simulink model "sm_car_"  (R2026b)
settings: Solver=ode23t  StopTime=100  MaxStep=0.4  AbsTol=1e-3  EnableMultiTasking=on
PreLoadFcn:
  | % Due to usability issue in Repeating Sequence block
  | warning('off','Simulink:Masking:Invalid');
  | 
  | % Eliminate unnecessary warnings in inactive variants
  | % Warnings generated only if you click through inactive variant
  | warning('off','MATLAB:nonExistentField');
  | warning('off','Simulink:Parameters:BlkParamUndefined');
PostLoadFcn:
  | set_param([bdroot '/Vehicle'],'popup_trailer','Off')
  | warning('off','sm:sli:setup:compile:LocalSolverNotSupported')
  | %sm_car_config_maneuver(bdroot,'WOT Braking');
  | sm_car_config_vehicle(bdroot,'false');
  | sm_car_config_logging(bdroot);
InitFcn:
  | sm_car_config_camera;
  | Vehicle = sm_car_vehcfg_checkConfig(Vehicle);
  | sm_car_check_tire_model(bdroot);
StartFcn:
  | tic;
StopFcn:
  | Elapsed_Sim_Time = toc;
  | % disp(['Elapsed Sim Time = ' num2str(Elapsed_Sim_Time)]);
undefined symbols (not defined in the file or in its folder): acc_theta, accel_ramp_rate, Axle1D, AxleIn, Camera, Control, Driver, Init, Maneuver, Pedal, Scene, ShaftL1, ShaftL2, ShaftR1, ShaftR2, Visual, X, xy_data_car_side, Y, Z
libraries: sm_lib x290, fl_lib x171, nesl_utility x144, simulink x60, simulink_extras x14, sdl_lib x14, SimscapeFluids_lib x7, Damper_Element x4, Tire_1x2x x4, ee_lib x3, Scene_Utilities x3, sharedTrackingLibrary x2
(part 11 of 22)

== system sm_car_/World/Scene/CRG Hockenheim F/STL Geometry Road ==
  Geometry : sm_lib/Body Elements/File Solid  ExtGeomFileName=CRG_Hockenheim_f.stl  UnitType=Custom  ExtGeomFileUnits=m  StepReaderType=HEX  ExportConvexHullGeometry=off  InertiaType=Custom  BasedOnType=DensityFromFile  Density=1000  DensityUnits=kg/m^3  Mass=1  MassUnits=kg  CenterOfMass=[0 0 0]  CenterOfMassUnits=m  MomentsOfInertia=[1 1 1]  MomentsOfInertiaUnits=kg*m^2  ProductsOfInertia=[0 0 0]  ProductsOfInertiaUnits=kg*m^2  GraphicType=FromGeometry  MarkerShape=Sphere  MarkerSize=10  GraphicVisPropType=SimpleVisualProperties  GraphicDiffuseColor=stl_clr  GraphicOpacity=stl_opc  GraphicSpecularColor=[0.5 0.5 0.5 1.0]  GraphicAmbientColor=[0.15 0.15 0.15 1.0]  GraphicEmissiveColor=[0.0 0.0 0.0 1.0]  GraphicShininess=75  DoExposeReferenceFrame=on  SerializedFrames=<Frames/>
  Transform Geometry : sm_lib/Frames and Transforms/Rigid Transform  RotationMethod=RotationSequence  FollAlignAxisA=+X  BaseAlignAxisA=+Y  FollAlignAxisB=+Y  BaseAlignAxisB=+Z  RotationStandardAxis=+Z  RotationAngle=0  RotationAngleUnits=rad  RotationArbitraryAxis=[0 0 1]  RotationSequenceAxes=FollowerAxes  RotationSequence=ZYX  RotationSequenceAngles=[stl_yaw stl_pitch stl_roll]  RotationSequenceAnglesUnits=rad  RotationMatrix=[1 0 0; 0 1 0; 0 0 1]  Quaternion=[1 0 0 0]  TranslationMethod=Cartesian  TranslationCartesianOffset=[stl_x stl_y stl_z]  TranslationCartesianOffsetUnits=m  TranslationStandardAxis=+Z  TranslationStandardOffset=0  TranslationStandardOffsetUnits=m  TranslationROffset=0  TranslationROffsetUnits=m  TranslationThetaOffset=0  TranslationThetaOffsetUnits=deg  TranslationZOffset=0  TranslationZOffsetUnits=m
  W : PMIOPort  Side=Right
  connections:
  Geometry/RConn1 -- Transform Geometry/RConn1
  Transform Geometry/LConn1 -- W/RConn1

== system sm_car_/World/Scene/Plane Grid/Grid ==
  Mesh Lines x : Subsystem  mask(Rectangular Mesh){mesh_lenx=grid_x, mesh_leny=grid_y, mesh_hx=hole_wy, mesh_hy=hole_ly, mesh_numhx=1, mesh_numhy=grid_num_sq_y, mesh_thickness=grid_z, mesh_rho=7000, mesh_color=grid_clr, mesh_opc=grid_opc}
      mask prompts: mesh_thickness "Thickness (m)"; mesh_rho "Density (kg/m^3)"; mesh_color "Color [RGB]"; mesh_opc "Opacity (0-1)"
      mask help: Rectangular mesh. Define outer dimensions, dimensions of holes, and thickness. R port is at the CG. Thickness defines the distance of the F frame from the B frame along the z-axis.
      mask init:
      | mesh_xsec = Extr_Data_Mesh(mesh_lenx, mesh_leny, mesh_numhx, mesh_numhy, mesh_hx, mesh_hy);
      mask DialogControl Control12 Prompt: Plot Profile
      mask DialogControl Control12 Callback:
      | v = get_param(gcb,'MaskWSVariables');
      | getMaskValue = containers.Map({v.Name}',{v.Value}');
      | evalin('base',...
      |     sprintf('Extr_Data_Mesh(%s,%s,%s,%s,%s,%s,''%s'');',...
      |     num2str(getMaskValue('mesh_lenx')),...
      |     num2str(getMaskValue('mesh_leny')),...
      |     num2str(getMaskValue('mesh_numhx')),...
      |     num2str(getMaskValue('mesh_numhy')),...
      |     num2str(getMaskValue('mesh_hx')),...
      |     num2str(getMaskValue('mesh_hy')),'plot'));
      mask DialogControl Control7 Prompt: X
      mask DialogControl Control8 Prompt: Y
      mask DialogControl Control9 Prompt: Mesh Length (m)
      mask DialogControl Control11 Prompt: Hole Length (m)
      mask DialogControl Control10 Prompt: Number of Holes
      mask Display: image('Mesh_IMAGE.png');
  "Mesh Lines y " : Subsystem  mask(Rectangular Mesh){mesh_lenx=grid_x, mesh_leny=grid_y, mesh_hx=hole_lx, mesh_hy=hole_wx, mesh_numhx=grid_num_sq_x, mesh_numhy=1, mesh_thickness=grid_z, mesh_rho=7000, mesh_color=grid_clr, mesh_opc=grid_opc}
      mask prompts: mesh_thickness "Thickness (m)"; mesh_rho "Density (kg/m^3)"; mesh_color "Color [RGB]"; mesh_opc "Opacity (0-1)"
      mask help: Rectangular mesh. Define outer dimensions, dimensions of holes, and thickness. R port is at the CG. Thickness defines the distance of the F frame from the B frame along the z-axis.
      mask init:
      | mesh_xsec = Extr_Data_Mesh(mesh_lenx, mesh_leny, mesh_numhx, mesh_numhy, mesh_hx, mesh_hy);
      mask DialogControl Control12 Prompt: Plot Profile
      mask DialogControl Control12 Callback:
      | v = get_param(gcb,'MaskWSVariables');
      | getMaskValue = containers.Map({v.Name}',{v.Value}');
      | evalin('base',...
      |     sprintf('Extr_Data_Mesh(%s,%s,%s,%s,%s,%s,''%s'');',...
      |     num2str(getMaskValue('mesh_lenx')),...
      |     num2str(getMaskValue('mesh_leny')),...
      |     num2str(getMaskValue('mesh_numhx')),...
      |     num2str(getMaskValue('mesh_numhy')),...
      |     num2str(getMaskValue('mesh_hx')),...
      |     num2str(getMaskValue('mesh_hy')),'plot'));
      mask DialogControl Control7 Prompt: X
      mask DialogControl Control8 Prompt: Y
      mask DialogControl Control9 Prompt: Mesh Length (m)
      mask DialogControl Control11 Prompt: Hole Length (m)
      mask DialogControl Control10 Prompt: Number of Holes
      mask Display: image('Mesh_IMAGE.png');
  Reference Frame{,1..3} (4 alike) : sm_lib/Frames and Transforms/Reference Frame
  R : PMIOPort  Side=Left
  connections:
  Reference Frame3/RConn1 -- Mesh Lines x/RConn2
  "Mesh Lines y "/LConn1 -- Mesh Lines x/LConn1 -- R/RConn1
  "Mesh Lines y "/RConn1 -- Reference Frame/RConn1
  Reference Frame1/RConn1 -- "Mesh Lines y "/RConn2
  Reference Frame2/RConn1 -- Mesh Lines x/RConn1

== system sm_car_/World/Scene/Plane Grid/Ground Plane ==
  Floor : sm_lib/Body Elements/Brick Solid  BrickDimensions=[gp_l, gp_w, gp_h]  BrickDimensionsUnits=m  ExportEntireGeometry=off  InertiaType=CalculateFromGeometry  BasedOnType=Density  Density=1000  DensityUnits=kg/m^3  Mass=1  MassUnits=kg  CenterOfMass=[0 0 0]  CenterOfMassUnits=m  MomentsOfInertia=[1 1 1]  MomentsOfInertiaUnits=kg*m^2  ProductsOfInertia=[0 0 0]  ProductsOfInertiaUnits=kg*m^2  GraphicType=FromGeometry  MarkerShape=Sphere  MarkerSize=10  GraphicVisPropType=SimpleVisualProperties  GraphicDiffuseColor=gp_clr  GraphicOpacity=gp_opc  GraphicSpecularColor=[0.5 0.5 0.5 1.0]  GraphicAmbientColor=[0.15 0.15 0.15 1.0]  GraphicEmissiveColor=[0.0 0.0 0.0 1.0]  GraphicShininess=75  DoExposeReferenceFrame=off  SerializedFrames=<Frames><Frame><Id>Frame1</Id><Value><Name>F</Name><Origin><Source>GeometricFeature</Source><FeatureName>+z surface</FeatureName></Origin><PrimaryAxis><DefinedDirection>+Z</DefinedDirection><Source>ReferenceFrame</Source><SourceDirection>+Z</SourceDirection><FeatureName></FeatureName></PrimaryAxis><SecondaryAxis><DefinedDirection>+X</DefinedDirection><Source>ReferenceFrame</Source><SourceDirection>+X</SourceDirection><FeatureName></FeatureName></SecondaryAxis></Value></Frame></Frames>
  W : PMIOPort  Side=Right
  connections:
  Floor/LConn1 -- W/RConn1

== system sm_car_/World/Scene/Skidpad/Circle Inner L ==
  Solid : sm_lib/Body Elements/Extruded Solid  ExtrusionType=General  PolygonNumSides=3  PolygonOuterRadius=1  PolygonOuterRadiusUnits=m  ExportEntireGeometry=off  ExtrusionCrossSection=xy_data_circ  ExtrusionCrossSectionUnits=m  ExportConvexHullGeometry=off  ExtrusionLength=circ_h  ExtrusionLengthUnits=m  InertiaType=CalculateFromGeometry  BasedOnType=Density  Density=1000  DensityUnits=kg/m^3  Mass=1  MassUnits=kg  CenterOfMass=[0 0 0]  CenterOfMassUnits=m  MomentsOfInertia=[1 1 1]  MomentsOfInertiaUnits=kg*m^2  ProductsOfInertia=[1 1 1]  ProductsOfInertiaUnits=kg*m^2  GraphicType=FromGeometry  MarkerShape=Sphere  MarkerSize=10  GraphicVisPropType=SimpleVisualProperties  GraphicDiffuseColor=[1.0 1.0 0.8]  GraphicOpacity=1.0  GraphicSpecularColor=[0.5 0.5 0.5 1.0]  GraphicAmbientColor=[0.15 0.15 0.15 1.0]  GraphicEmissiveColor=[0.0 0.0 0.0 1.0]  GraphicShininess=75  DoExposeReferenceFrame=on  SerializedFrames=<Frames/>
  W : PMIOPort  Side=Right
  connections:
  Solid/RConn1 -- W/RConn1

== system sm_car_/World/Scene/Skidpad/Circle Inner R ==
  Solid : sm_lib/Body Elements/Extruded Solid  ExtrusionType=General  PolygonNumSides=3  PolygonOuterRadius=1  PolygonOuterRadiusUnits=m  ExportEntireGeometry=off  ExtrusionCrossSection=xy_data_circ  ExtrusionCrossSectionUnits=m  ExportConvexHullGeometry=off  ExtrusionLength=circ_h  ExtrusionLengthUnits=m  InertiaType=CalculateFromGeometry  BasedOnType=Density  Density=1000  DensityUnits=kg/m^3  Mass=1  MassUnits=kg  CenterOfMass=[0 0 0]  CenterOfMassUnits=m  MomentsOfInertia=[1 1 1]  MomentsOfInertiaUnits=kg*m^2  ProductsOfInertia=[1 1 1]  ProductsOfInertiaUnits=kg*m^2  GraphicType=FromGeometry  MarkerShape=Sphere  MarkerSize=10  GraphicVisPropType=SimpleVisualProperties  GraphicDiffuseColor=[1.0 1.0 0.8]  GraphicOpacity=1.0  GraphicSpecularColor=[0.5 0.5 0.5 1.0]  GraphicAmbientColor=[0.15 0.15 0.15 1.0]  GraphicEmissiveColor=[0.0 0.0 0.0 1.0]  GraphicShininess=75  DoExposeReferenceFrame=on  SerializedFrames=<Frames/>
  W : PMIOPort  Side=Right
  connections:
  Solid/RConn1 -- W/RConn1

== system sm_car_/World/Scene/Skidpad/Circle Outer L ==
  Solid : sm_lib/Body Elements/Extruded Solid  ExtrusionType=General  PolygonNumSides=3  PolygonOuterRadius=1  PolygonOuterRadiusUnits=m  ExportEntireGeometry=off  ExtrusionCrossSection=xy_data_circ  ExtrusionCrossSectionUnits=m  ExportConvexHullGeometry=off  ExtrusionLength=circ_h  ExtrusionLengthUnits=m  InertiaType=CalculateFromGeometry  BasedOnType=Density  Density=1000  DensityUnits=kg/m^3  Mass=1  MassUnits=kg  CenterOfMass=[0 0 0]  CenterOfMassUnits=m  MomentsOfInertia=[1 1 1]  MomentsOfInertiaUnits=kg*m^2  ProductsOfInertia=[1 1 1]  ProductsOfInertiaUnits=kg*m^2  GraphicType=FromGeometry  MarkerShape=Sphere  MarkerSize=10  GraphicVisPropType=SimpleVisualProperties  GraphicDiffuseColor=[1.0 1.0 0.8]  GraphicOpacity=1.0  GraphicSpecularColor=[0.5 0.5 0.5 1.0]  GraphicAmbientColor=[0.15 0.15 0.15 1.0]  GraphicEmissiveColor=[0.0 0.0 0.0 1.0]  GraphicShininess=75  DoExposeReferenceFrame=on  SerializedFrames=<Frames/>
  W : PMIOPort  Side=Right
  connections:
  Solid/RConn1 -- W/RConn1

== system sm_car_/World/Scene/Skidpad/Circle Outer R ==
  Solid : sm_lib/Body Elements/Extruded Solid  ExtrusionType=General  PolygonNumSides=3  PolygonOuterRadius=1  PolygonOuterRadiusUnits=m  ExportEntireGeometry=off  ExtrusionCrossSection=xy_data_circ  ExtrusionCrossSectionUnits=m  ExportConvexHullGeometry=off  ExtrusionLength=circ_h  ExtrusionLengthUnits=m  InertiaType=CalculateFromGeometry  BasedOnType=Density  Density=1000  DensityUnits=kg/m^3  Mass=1  MassUnits=kg  CenterOfMass=[0 0 0]  CenterOfMassUnits=m  MomentsOfInertia=[1 1 1]  MomentsOfInertiaUnits=kg*m^2  ProductsOfInertia=[1 1 1]  ProductsOfInertiaUnits=kg*m^2  GraphicType=FromGeometry  MarkerShape=Sphere  MarkerSize=10  GraphicVisPropType=SimpleVisualProperties  GraphicDiffuseColor=[1.0 1.0 0.8]  GraphicOpacity=1.0  GraphicSpecularColor=[0.5 0.5 0.5 1.0]  GraphicAmbientColor=[0.15 0.15 0.15 1.0]  GraphicEmissiveColor=[0.0 0.0 0.0 1.0]  GraphicShininess=75  DoExposeReferenceFrame=on  SerializedFrames=<Frames/>
  W : PMIOPort  Side=Right
  connections:
  Solid/RConn1 -- W/RConn1

== system sm_car_/World/Scene/Skidpad/Ground Plane ==
  Floor : sm_lib/Body Elements/Brick Solid  BrickDimensions=[gp_l, gp_w, gp_h]  BrickDimensionsUnits=m  ExportEntireGeometry=off  InertiaType=CalculateFromGeometry  BasedOnType=Density  Density=1000  DensityUnits=kg/m^3  Mass=1  MassUnits=kg  CenterOfMass=[0 0 0]  CenterOfMassUnits=m  MomentsOfInertia=[1 1 1]  MomentsOfInertiaUnits=kg*m^2  ProductsOfInertia=[0 0 0]  ProductsOfInertiaUnits=kg*m^2  GraphicType=FromGeometry  MarkerShape=Sphere  MarkerSize=10  GraphicVisPropType=SimpleVisualProperties  GraphicDiffuseColor=gp_clr  GraphicOpacity=gp_opc  GraphicSpecularColor=[0.5 0.5 0.5 1.0]  GraphicAmbientColor=[0.15 0.15 0.15 1.0]  GraphicEmissiveColor=[0.0 0.0 0.0 1.0]  GraphicShininess=75  DoExposeReferenceFrame=off  SerializedFrames=<Frames><Frame><Id>Frame1</Id><Value><Name>F</Name><Origin><Source>GeometricFeature</Source><FeatureName>+z surface</FeatureName></Origin><PrimaryAxis><DefinedDirection>+Z</DefinedDirection><Source>ReferenceFrame</Source><SourceDirection>+Z</SourceDirection><FeatureName></FeatureName></PrimaryAxis><SecondaryAxis><DefinedDirection>+X</DefinedDirection><Source>ReferenceFrame</Source><SourceDirection>+X</SourceDirection><FeatureName></FeatureName></SecondaryAxis></Value></Frame></Frames>
  W : PMIOPort  Side=Right
  connections:
  Floor/LConn1 -- W/RConn1

== system sm_car_/Controller/Default/State Estimation/Sensor Noise Simulation/noise a_x ==
  <w> : Inport
  Add2 : Sum
  Band-Limited White Noise2 : simulink/Sources/Band-Limited White Noise  Cov=[1.22e-4]  Ts=0.01  seed=[512361]
  Quantizer2 : Quantizer  QuantizationInterval=0.0047
  Zero-Order Hold2 : ZeroOrderHold  SampleTime=0.01
  a_x_n : Outport
  wires:
  Add2/1 -> a_x_n/1  "a_x_n"
  <w>/1 -> Quantizer2/1
  Zero-Order Hold2/1 -> Add2/1
  Band-Limited White Noise2/1 -> Add2/2
  Quantizer2/1 -> Zero-Order Hold2/1

== system sm_car_/Controller/Default/State Estimation/Sensor Noise Simulation/noise a_y ==
  <w> : Inport
  Add2 : Sum
  Band-Limited White Noise2 : simulink/Sources/Band-Limited White Noise  Cov=[1.22e-4]  Ts=0.01  seed=[092756]
  Quantizer2 : Quantizer  QuantizationInterval=0.0047
  Zero-Order Hold2 : ZeroOrderHold  SampleTime=0.01
  a_y_n : Outport
  wires:
  Add2/1 -> a_y_n/1  "a_y_n"
  <w>/1 -> Quantizer2/1
  Zero-Order Hold2/1 -> Add2/1
  Band-Limited White Noise2/1 -> Add2/2
  Quantizer2/1 -> Zero-Order Hold2/1

== system sm_car_/Controller/Default/State Estimation/Sensor Noise Simulation/noise omega_fl ==
  <w> : Inport
  Add2 : Sum
  Band-Limited White Noise2 : simulink/Sources/Band-Limited White Noise  Cov=[1e-4]  Ts=0.01  seed=[12451]
  Quantizer2 : Quantizer  QuantizationInterval=2 * pi / 25
  Zero-Order Hold2 : ZeroOrderHold  SampleTime=0.01
  omega_rl : Outport
  wires:
  Add2/1 -> omega_rl/1  "omega_rl"
  <w>/1 -> Quantizer2/1
  Zero-Order Hold2/1 -> Add2/1
  Band-Limited White Noise2/1 -> Add2/2
  Quantizer2/1 -> Zero-Order Hold2/1

== system sm_car_/Controller/Default/State Estimation/Sensor Noise Simulation/noise omega_fr ==
  <w> : Inport
  Add3 : Sum
  Band-Limited White Noise3 : simulink/Sources/Band-Limited White Noise  Cov=[1e-4]  Ts=0.01  seed=[68595]
  Quantizer3 : Quantizer  QuantizationInterval=2 * pi / 25
  Zero-Order Hold3 : ZeroOrderHold  SampleTime=0.01
  omega_rr : Outport
  wires:
  Add3/1 -> omega_rr/1  "omega_rr"
  Band-Limited White Noise3/1 -> Add3/2
  Zero-Order Hold3/1 -> Add3/1
  <w>/1 -> Quantizer3/1
  Quantizer3/1 -> Zero-Order Hold3/1

== system sm_car_/Controller/Default/State Estimation/Sensor Noise Simulation/noise omega_rl ==
  <w> : Inport
  Add : Sum
  Band-Limited White Noise : simulink/Sources/Band-Limited White Noise  Cov=[1e-4]  Ts=0.01  seed=[23341]
  Quantizer : Quantizer  QuantizationInterval=2 * pi / 94
  Zero-Order Hold : ZeroOrderHold  SampleTime=0.01
  omega_rl : Outport
  wires:
  Quantizer/1 -> Zero-Order Hold/1
  <w>/1 -> Quantizer/1
  Band-Limited White Noise/1 -> Add/2
  Add/1 -> omega_rl/1  "omega_rl"
  Zero-Order Hold/1 -> Add/1

== system sm_car_/Controller/Default/State Estimation/Sensor Noise Simulation/noise omega_rr ==
  <w> : Inport
  Add1 : Sum
  Band-Limited White Noise1 : simulink/Sources/Band-Limited White Noise  Cov=[1e-4]  Ts=0.01  seed=[41245]
  Quantizer1 : Quantizer  QuantizationInterval=2 * pi / 94
  Zero-Order Hold1 : ZeroOrderHold  SampleTime=0.01
  omega_rr : Outport
  wires:
  Add1/1 -> omega_rr/1  "omega_rr"
  Quantizer1/1 -> Zero-Order Hold1/1
  <w>/1 -> Quantizer1/1
  Band-Limited White Noise1/1 -> Add1/2
  Zero-Order Hold1/1 -> Add1/1

== system sm_car_/Controller/Default/State Estimation/Sensor Noise Simulation/noise v_gps ==
  <vx> : Inport
  <vy> : Inport  Port=2
  <vz> : Inport  Port=3
  Add : Sum  Inputs=+++
  Add2 : Sum
  Band-Limited White Noise2 : simulink/Sources/Band-Limited White Noise  Cov=[9e-4]  Ts=0.1  seed=[645743]
  Quantizer2 : Quantizer  QuantizationInterval=0.01
  Sqrt : Sqrt
  Square : Math  Operator=square
  Square1 : Math  Operator=square
  Square2 : Math  Operator=square
  Zero-Order Hold2 : ZeroOrderHold  SampleTime=0.1
  V_n : Outport
  wires:
  Quantizer2/1 -> Zero-Order Hold2/1
  Band-Limited White Noise2/1 -> Add2/2
  Zero-Order Hold2/1 -> Add2/1
  <vx>/1 -> Square/1
  Add2/1 -> V_n/1  "V_n"
  Square/1 -> Add/1
  <vy>/1 -> Square1/1
  <vz>/1 -> Square2/1
  Square1/1 -> Add/2
  Square2/1 -> Add/3
  Add/1 -> Sqrt/1
  Sqrt/1 -> Quantizer2/1

== system sm_car_/Controller/Default/State Estimation/Sensor Noise Simulation/noise yaw rate ==
  <w> : Inport
  Add2 : Sum
  Band-Limited White Noise2 : simulink/Sources/Band-Limited White Noise  Cov=[7.29e-7]  Ts=0.01  seed=[809953]
  Quantizer2 : Quantizer  QuantizationInterval=0.001
  Zero-Order Hold2 : ZeroOrderHold  SampleTime=0.01
  nYaw_n : Outport
  wires:
  Quantizer2/1 -> Zero-Order Hold2/1
  Band-Limited White Noise2/1 -> Add2/2
  Zero-Order Hold2/1 -> Add2/1
  <w>/1 -> Quantizer2/1
  Add2/1 -> nYaw_n/1  "nYaw_n"

== system sm_car_/Controller/TrqVec 4Motor/Brake Control/ABS/Calculate Slip ==
  WhlSpd : Inport
  VehSpdEst : Inport  Port=2
  Abs : Abs  ZeroCross=off  SaturateOnIntegerOverflow=off
  Bus Creator : BusCreator  Inputs=4
  Bus Selector1 : BusSelector  OutputSignals=L1.v,R1.v,L2.v,R2.v
  Constant : Constant
  Demux : Demux
  Fcn{,1..3} (4 alike) : Fcn  Expr=abs(u(1)*u(2)-u(3))/u(3)
  Mux{,1..3} (4 alike) : Mux  Inputs=3
  Mux4 : Mux
  Mux5 : Mux
  Product : Product
  Saturation : Saturate  UpperLimit=inf  LowerLimit=eps  ZeroCross=off
  Saturation1 : Saturate  UpperLimit=1  LowerLimit=0
  Sign : Signum  ZeroCross=off
  Wheel Speeds and Slip : Scope  NumInputPorts=2
      settings: ActiveDisplayYMinimum=-11.64241  ActiveDisplayYMaximum=114.01232  DataLoggingVariableName=ScopeData2
  Slip : Outport  VectorParamsAs1DForOutWhenUnconnected=off
  wires:
  WhlSpd/1 -> Bus Selector1/1
  Bus Selector1/2 -> Mux4/2, Mux1/2  "<v>"
  Bus Selector1/4 -> Mux4/4, Mux3/2  "<v>"
  Bus Selector1/1 -> Mux4/1, Mux/2  "<v>"
  Bus Selector1/3 -> Mux4/3, Mux2/2  "<v>"
  Constant/1 -> Mux/1, Mux1/1, Mux3/1, Mux2/1
  VehSpdEst/1 -> Sign/1, Abs/1
  Demux/1 -> Bus Creator/1  "L1"
  Demux/2 -> Bus Creator/2  "R1"
  Demux/3 -> Bus Creator/3  "L2"
  Demux/4 -> Bus Creator/4  "R2"
  Bus Creator/1 -> Wheel Speeds and Slip/2, Slip/1  "Slip"
  Product/1 -> Mux3/3, Mux2/3, Mux1/3, Mux/3
  Abs/1 -> Saturation/1
  Saturation/1 -> Product/1
  Sign/1 -> Product/2
  Mux/1 -> Fcn/1
  Mux1/1 -> Fcn1/1
  Mux2/1 -> Fcn2/1
  Mux3/1 -> Fcn3/1
  Mux4/1 -> Wheel Speeds and Slip/1  "Wheel Speeds"
  Mux5/1 -> Saturation1/1
  Saturation1/1 -> Demux/1
  Fcn/1 -> Mux5/1  "L1"
  Fcn1/1 -> Mux5/2  "R1"
  Fcn2/1 -> Mux5/3  "L2"
  Fcn3/1 -> Mux5/4  "R2"

== system sm_car_/Controller/TrqVec 4Motor/Brake Control/ABS/Sensor ==
  Body : Inport
  WhlSpd : Inport  Port=2
  Bus Creator{,3..5} (4 alike) : BusCreator  Inputs=1
  Bus Creator6 : BusCreator  Inputs=5
  Bus Selector : BusSelector  OutputSignals=vx,vy  OutputAsBus=on
  Bus Selector4 : BusSelector  OutputSignals=WhlL1.n,WhlR1.n,WhlL2.n,WhlR2.n,WhlL2.qxyz
  Gain : Gain  Gain=3.6*abs_tire_radiusF
  Gain1 : Gain  Gain=3.6*abs_tire_radiusF
  Gain2 : Gain  Gain=3.6*abs_tire_radiusR
  Gain3 : Gain  Gain=3.6*abs_tire_radiusR
  Gain4 : Gain  Gain=3.6
  Terminator1 : Terminator  Commented=on
  Vel in xy plane : Fcn  Expr=sqrt(u(1)^2+u(2)^2)
  missing tooth : Subsystem  Commented=on
  GroundSpd : Outport  VectorParamsAs1DForOutWhenUnconnected=off
  wires:
  Gain1/1 -> Bus Creator3/1  "v"
  missing tooth/1(Out1) -> Terminator1/1  "v"
  Gain2/1 -> Bus Creator4/1  "v"
  Bus Selector4/5 -> missing tooth/2(<qxyz>)  "<qxyz>"
  Bus Creator5/1 -> Bus Creator6/5  "R2"
  Gain3/1 -> Bus Creator5/1  "v"
  Bus Creator/1 -> Bus Creator6/2  "L1"
  Bus Selector4/2 -> Gain1/1  "<n>"
  Bus Creator4/1 -> Bus Creator6/4  "L2"
  Bus Selector4/3 -> Gain2/1, missing tooth/1(<omega>)  "<n>"
  Gain/1 -> Bus Creator/1  "v"
  Body/1 -> Bus Selector/1
  Bus Creator3/1 -> Bus Creator6/3  "R1"
  Gain4/1 -> Bus Creator6/1  "v"
  Bus Selector4/1 -> Gain/1  "<n>"
  Bus Selector4/4 -> Gain3/1  "<n>"
  WhlSpd/1 -> Bus Selector4/1
  Bus Creator6/1 -> GroundSpd/1
  Vel in xy plane/1 -> Gain4/1  "speed"
  Bus Selector/1 -> Vel in xy plane/1

== system sm_car_/Controller/TrqVec 4Motor/Brake Control/ABS/Valve Control L1 ==
  Slip : Inport
  vSpdEst : Inport  Port=2
  Categorize Surface : Subsystem
  Code to Valves : Subsystem
  Demux : Demux  Outputs=2
  Logic : Stateflow chart  TreatAsAtomicUnit=on
  Mux : Mux  Inputs=2
  Product : Product
  Subsystem : Subsystem
  Subsystem1 : Subsystem
  Valve : Outport  VectorParamsAs1DForOutWhenUnconnected=off
  wires:
  Logic/1(Mod_State) -> Categorize Surface/1(Mod State), Code to Valves/1(C)
  Logic/2(Mod_Dur) -> Product/2
  Slip/1 -> Logic/1(Slip)
  Code to Valves/1(V) -> Product/1
  vSpdEst/1 -> Logic/2(vSpdEst)
  Product/1 -> Demux/1
  Demux/1 -> Subsystem/1(OnT)
  Demux/2 -> Subsystem1/1(OnT)
  Mux/1 -> Valve/1
  Subsystem/1(vSig) -> Mux/1, Categorize Surface/2(Apply Valve)
  Subsystem1/1(vSig) -> Mux/2

== system sm_car_/Controller/TrqVec 4Motor/Brake Control/ABS/Valve Control L2 ==
  Slip : Inport
  vSpdEst : Inport  Port=2
  Categorize Surface : Subsystem
  Code to Valves : Subsystem
  Demux : Demux  Outputs=2
  Logic : Stateflow chart  TreatAsAtomicUnit=on
  Mux : Mux  Inputs=2
  Product : Product
  Subsystem : Subsystem
  Subsystem1 : Subsystem
  Valve : Outport  VectorParamsAs1DForOutWhenUnconnected=off
  wires:
  Logic/1(Mod_State) -> Categorize Surface/1(Mod State), Code to Valves/1(C)
  Logic/2(Mod_Dur) -> Product/2
  Slip/1 -> Logic/1(Slip)
  Code to Valves/1(V) -> Product/1
  vSpdEst/1 -> Logic/2(vSpdEst)
  Product/1 -> Demux/1
  Demux/1 -> Subsystem/1(OnT)
  Demux/2 -> Subsystem1/1(OnT)
  Mux/1 -> Valve/1
  Subsystem/1(vSig) -> Mux/1, Categorize Surface/2(Apply Valve)
  Subsystem1/1(vSig) -> Mux/2

== system sm_car_/Controller/TrqVec 4Motor/Brake Control/ABS/Valve Control R1 ==
  Slip : Inport
  vSpdEst : Inport  Port=2
  Categorize Surface : Subsystem
  Code to Valves : Subsystem
  Demux : Demux  Outputs=2
  Logic : Stateflow chart  TreatAsAtomicUnit=on
  Mux : Mux  Inputs=2
  Product : Product
  Subsystem : Subsystem
  Subsystem1 : Subsystem
  Valve : Outport  VectorParamsAs1DForOutWhenUnconnected=off
  wires:
  Logic/1(Mod_State) -> Categorize Surface/1(Mod State), Code to Valves/1(C)
  Logic/2(Mod_Dur) -> Product/2
  Slip/1 -> Logic/1(Slip)
  Code to Valves/1(V) -> Product/1
  vSpdEst/1 -> Logic/2(vSpdEst)
  Product/1 -> Demux/1
  Demux/1 -> Subsystem/1(OnT)
  Demux/2 -> Subsystem1/1(OnT)
  Mux/1 -> Valve/1
  Subsystem/1(vSig) -> Mux/1, Categorize Surface/2(Apply Valve)
  Subsystem1/1(vSig) -> Mux/2

== system sm_car_/Controller/TrqVec 4Motor/Brake Control/ABS/Valve Control R2 ==
  Slip : Inport
  vSpdEst : Inport  Port=2
  Categorize Surface : Subsystem
  Code to Valves : Subsystem
  Demux : Demux  Outputs=2
  Logic : Stateflow chart  TreatAsAtomicUnit=on
  Mux : Mux  Inputs=2
  Product : Product
  Subsystem : Subsystem
  Subsystem1 : Subsystem
  Valve : Outport  VectorParamsAs1DForOutWhenUnconnected=off
  wires:
  Logic/1(Mod_State) -> Categorize Surface/1(Mod State), Code to Valves/1(C)
  Logic/2(Mod_Dur) -> Product/2
  Slip/1 -> Logic/1(Slip)
  Code to Valves/1(V) -> Product/1
  vSpdEst/1 -> Logic/2(vSpdEst)
  Product/1 -> Demux/1
  Demux/1 -> Subsystem/1(OnT)
  Demux/2 -> Subsystem1/1(OnT)
  Mux/1 -> Valve/1
  Subsystem/1(vSig) -> Mux/1, Categorize Surface/2(Apply Valve)
  Subsystem1/1(vSig) -> Mux/2

== system sm_car_/Controller/TrqVec 4Motor/Brake Control/ABS/Vehicle Speed ==
  Sensors : Inport
  Bus Selector : BusSelector  OutputSignals=v
  vSpdEst : Outport  VectorParamsAs1DForOutWhenUnconnected=off
  wires:
  Sensors/1 -> Bus Selector/1
  Bus Selector/1 -> vSpdEst/1  "<v>"

== system sm_car_/Controller/TrqVec 4Motor/Power_TqVec/Torque Vectoring/Accel Torque Request ==
  note: Assumes both rear motors have same torque speed curve
  MotSpdL2 : Inport
  MotSpdR2 : Inport  Port=2
  MaxMotTrqVsSpdA1 : Lookup_n-D  NumberOfTableDimensions=1  BreakpointsForDimension1=Control.MotorL2.TorqueSpd.w.Value  Table=Control.MotorL2.TorqueSpd.trq.Value  ExtrapMethod=Clip  UseLastTableValue=on  InternalRulePriority=Speed  OutDataTypeStr=Inherit: Inherit from 'Table data'  RndMeth=Simplest
  Terminator : Terminator
  rads_to_rpm : Gain  Gain=30/pi
  rads_to_rpm1 : Gain  Gain=30/pi
  TrqMax : Outport  VectorParamsAs1DForOutWhenUnconnected=off
  wires:
  rads_to_rpm1/1 -> Terminator/1
  MotSpdR2/1 -> rads_to_rpm1/1
  MaxMotTrqVsSpdA1/1 -> TrqMax/1
  MotSpdL2/1 -> rads_to_rpm/1
  rads_to_rpm/1 -> MaxMotTrqVsSpdA1/1

== system sm_car_/Controller/TrqVec 4Motor/Power_TqVec/Torque Vectoring/Enable ==
  note: Ramp up amount of torque vectoring over a range.
  note: Steer angle threshold to enable torque vectoring
  vx : Inport
  aSteerWheel : Inport  Port=2
  Abs : Abs  ZeroCross=off  SaturateOnIntegerOverflow=off
  Data Type Conversion : DataTypeConversion  OutDataTypeStr=double  SaturateOnIntegerOverflow=off  RndMeth=Floor
  Divide : Product  Inputs=*/
  Enable vx : simulink/Logic and Bit Operations/Compare To Constant  relop=>  const=vx_enable  OutDataTypeStr=boolean  ZeroCross=off
  Gain : Gain  Gain=0.25
  Product : Product
  Saturation : Saturate  UpperLimit=1  LowerLimit=0  ZeroCross=off
  Subtract : Sum  Inputs=+-
  const : Constant  Value=aSteerWheel_enable
  Enable : Outport  VectorParamsAs1DForOutWhenUnconnected=off
  wires:
  Gain/1 -> Divide/1
  Product/1 -> Enable/1
  Divide/1 -> Saturation/1
  Subtract/1 -> Gain/1
  Abs/1 -> Subtract/1
  Saturation/1 -> Product/2
  Data Type Conversion/1 -> Product/1
  Enable vx/1 -> Data Type Conversion/1
  const/1 -> Subtract/2, Divide/2
  aSteerWheel/1 -> Abs/1
  vx/1 -> Enable vx/1

== system sm_car_/Controller/TrqVec 4Motor/Power_TqVec/Torque Vectoring/Vehicle Slip Angle Error ==
  vx : Inport
  aSteerWheel : Inport  Port=2
  nYaw : Inport  Port=3
  Add1 : Sum  Inputs=-+
  Distance Yaw Ctr Front Axle : Constant  Value=Vehicle.Chassis.Body.sAxle2.Value(1)/(-2)
  Divide3 : Product  Inputs=*/
  Multiply2 : Product
  Mux : Mux  Inputs=2
  Scope : Scope  NumInputPorts=2
      settings: ActiveDisplayYMinimum=-0.04829  ActiveDisplayYMaximum=0.00545
  Steering Wheel to Driving Wheel : Gain  Gain=aStr_to_aWhl
  Error : Outport  VectorParamsAs1DForOutWhenUnconnected=off
  wires:
  Mux/1 -> Scope/1
  Multiply2/1 -> Divide3/1
  Steering Wheel to Driving Wheel/1 -> Mux/2, Add1/2  "Wheel Angle"
  Distance Yaw Ctr Front Axle/1 -> Multiply2/1
  aSteerWheel/1 -> Steering Wheel to Driving Wheel/1
  nYaw/1 -> Multiply2/2
  Add1/1 -> Scope/2, Error/1  "Error"
  vx/1 -> Divide3/2
  Divide3/1 -> Add1/1, Mux/1  "Vehicle Slip Angle"

== system sm_car_/Controller/TrqVec_FLC_V3/Power Control/State Estimation/Sensor Noise Simulation ==
  <vx> : Inport
  <vy> : Inport  Port=2
  <vz> : Inport  Port=3
  <nYaw> : Inport  Port=4
  <gx> : Inport  Port=5
  <gy> : Inport  Port=6
  <w_fl> : Inport  Port=7
  <w_fr> : Inport  Port=8
  <w_rl> : Inport  Port=9
  <w_rr> : Inport  Port=10
  delta : Inport  Port=11
  Bus Creator : BusCreator  Inputs=5
  Bus Creator1 : BusCreator  Inputs=4
  Data Type Conversion{,3..10} (9 alike) : DataTypeConversion  OutDataTypeStr=single  SaturateOnIntegerOverflow=off  RndMeth=Floor
  noise a_x : Subsystem
  noise a_y : Subsystem
  noise omega_fl : Subsystem
  noise omega_fr : Subsystem
  noise omega_rl : Subsystem
  noise omega_rr : Subsystem
  noise v_gps : Subsystem
  noise yaw rate : Subsystem
  Inputs : Outport
  Meas : Outport  Port=2
  wires:
  <vz>/1 -> noise v_gps/3(<vz>)
  <vy>/1 -> noise v_gps/2(<vy>)
  noise v_gps/1(V_n) -> Data Type Conversion/1
  Data Type Conversion10/1 -> Bus Creator/5  "omega_rr_n"
  Data Type Conversion9/1 -> Bus Creator/4  "omega_rl_n"
  Data Type Conversion8/1 -> Bus Creator/1  "delta"
  Data Type Conversion7/1 -> Bus Creator/3  "omega_fr_n"
  Data Type Conversion6/1 -> Bus Creator/2  "omega_fl_n"
  Data Type Conversion5/1 -> Bus Creator1/4  "a_y_n"
  Data Type Conversion4/1 -> Bus Creator1/3  "a_x_n"
  Data Type Conversion3/1 -> Bus Creator1/2  "nYaw_n"
  Data Type Conversion/1 -> Bus Creator1/1  "V_GPS_n"
  Bus Creator1/1 -> Meas/1
  noise omega_fr/1(omega_rr) -> Data Type Conversion7/1
  <w_rr>/1 -> noise omega_rr/1(<w>)
  noise omega_rr/1(omega_rr) -> Data Type Conversion10/1
  <gy>/1 -> noise a_y/1(<w>)
  <w_rl>/1 -> noise omega_rl/1(<w>)
  noise yaw rate/1(nYaw_n) -> Data Type Conversion3/1
  noise omega_rl/1(omega_rl) -> Data Type Conversion9/1
  Bus Creator/1 -> Inputs/1
  noise a_y/1(a_y_n) -> Data Type Conversion5/1
  noise omega_fl/1(omega_rl) -> Data Type Conversion6/1
  <vx>/1 -> noise v_gps/1(<vx>)
  noise a_x/1(a_x_n) -> Data Type Conversion4/1
  <gx>/1 -> noise a_x/1(<w>)
  <w_fr>/1 -> noise omega_fr/1(<w>)
  <nYaw>/1 -> noise yaw rate/1(<w>)
  <w_fl>/1 -> noise omega_fl/1(<w>)
  delta/1 -> Data Type Conversion8/1

== system sm_car_/Controller/TrqVec_FLC_V3/Power Control/State Estimation/UKF ==
  StateTransitionFcnInputs : Inport  PortDimensions=5
  y1 : Inport  Port=2
  Compare To Constant : simulink/Logic and Bit Operations/Compare To Constant  relop=<=  const=0.5  OutDataTypeStr=boolean
  Constant : Constant  Value=0  OutDataTypeStr=single  SampleTime=0.003
  Constant1 : Constant  Value=0  OutDataTypeStr=single
  Delay : Delay  DelayLength=1  SampleTime=0.003
  Demux : Demux  Outputs=5
  MATLAB Function : MATLAB Function  TreatAsAtomicUnit=on
  Mux : Mux  Inputs=5
  Switch : Switch  Criteria=u2 ~= 0  SaturateOnIntegerOverflow=off  InputSameDT=off
  Unscented Kalman Filter : sharedTrackingLibrary/Unscented Kalman Filter  StateTransitionFcn=prediction_model  HasAdditiveProcessNoise=Additive  ProcessNoise=diag([1e-5, 8e-6, 1e-6, 5e-5, 1e-4])  HasTimeVaryingProcessNoise=on  HasStateTransitionFcnExtraArgument=1  InitialState=[0.4; 0; 0; 0; 0]  InitialStateCovariance=diag([0.04, 0.04, 1e-3, 0.1, 0.1])  Alpha=0.1  Beta=2  Kappa=0  MeasurementFcn1=measurement_model  HasMeasurementEnablePort1=off  HasAdditiveMeasurementNoise1=Additive  MeasurementNoise1=[9e-4, 7.29e-7, 1.22e-4, 1.22e-4]  HasTimeVaryingMeasurementNoise1=off  HasMeasurementFcnExtraArgument1=1  HasMeasurementWrapping1=on  MeasurementFcn2=myMeasurementFcn  HasMeasurementEnablePort2=off  HasAdditiveMeasurementNoise2=Additive  MeasurementNoise2=1  HasTimeVaryingMeasurementNoise2=off  HasMeasurementFcnExtraArgument2=0  HasMeasurementWrapping2=off  MeasurementFcn3=myMeasurementFcn  HasMeasurementEnablePort3=off  HasAdditiveMeasurementNoise3=Additive  MeasurementNoise3=1  HasTimeVaryingMeasurementNoise3=off  HasMeasurementFcnExtraArgument3=0  HasMeasurementWrapping3=off  MeasurementFcn4=myMeasurementFcn  HasMeasurementEnablePort4=off  HasAdditiveMeasurementNoise4=Additive  MeasurementNoise4=1  HasTimeVaryingMeasurementNoise4=off  HasMeasurementFcnExtraArgument4=0  HasMeasurementWrapping4=off  MeasurementFcn5=myMeasurementFcn  HasMeasurementEnablePort5=off  HasAdditiveMeasurementNoise5=Additive  MeasurementNoise5=1  HasTimeVaryingMeasurementNoise5=off  HasMeasurementFcnExtraArgument5=0  HasMeasurementWrapping5=off  EnableMultirate=off  StateTransitionFcnSampleTime=1  MeasurementFcn1SampleTime=1  MeasurementFcn2SampleTime=1  MeasurementFcn3SampleTime=1  MeasurementFcn4SampleTime=1  MeasurementFcn5SampleTime=1  UseCurrentEstimator=on  OutputStateCovariance=off  DataType=single  SampleTime=0.003  NumberOfMeasurements=1
      settings: LibrarySourceBlock=cstblocks/State Estimation/Unscented Kalman Filter
  xhat : Outport
  wires:
  Mux/1 -> xhat/1
  Demux/5 -> Mux/5
  Demux/4 -> Mux/4
  Demux/3 -> Mux/3
  Switch/1 -> Mux/2
  Demux/2 -> Switch/3
  Demux/1 -> Compare To Constant/1, Mux/1
  Constant1/1 -> Switch/1
  Compare To Constant/1 -> Switch/2
  Delay/1 -> MATLAB Function/1(xhat)
  MATLAB Function/1(Q) -> Unscented Kalman Filter/1
  Unscented Kalman Filter/1 -> Demux/1, Delay/1
  Constant/1 -> Unscented Kalman Filter/4
  StateTransitionFcnInputs/1 -> Unscented Kalman Filter/2
  y1/1 -> Unscented Kalman Filter/3

== system sm_car_/Driver/Closed Loop/Maneuver/Count Lap/Triggered Subsystem ==
  Up Down : Inport
  Trigger : TriggerPort  VariantControl=Variant  ZeroCross=off
  Memory : Memory  InheritSampleTime=on
  Sum : Sum  Inputs=|++
  Num Laps : Outport  VectorParamsAs1DForOutWhenUnconnected=off
  wires:
  Memory/1 -> Sum/1
  Sum/1 -> Memory/1, Num Laps/1
  Up Down/1 -> Sum/2

== system sm_car_/Driver/Closed Loop/Maneuver/PoseTargetVisual/Count Lap ==
  note: If on the previous step, the vehicle was in the last 5 percent of the trajectory and now it is on the first 5 percent of the trajectory, increment the number of laps.
  note: If on the previous step, the vehicle was in the first 5 percent of the trajectory and now it is on the last 5 percent of the trajectory, decrement the number of laps.
  ad : Inport
  AND Add Lap : Logic  IconShape=distinctive  AllPortsSameDT=off  OutDataTypeStr=boolean
  AND Subtract Lap : Logic  IconShape=distinctive  AllPortsSameDT=off  OutDataTypeStr=boolean
  Data Type Conversion : DataTypeConversion  SaturateOnIntegerOverflow=off  RndMeth=Floor
  Data Type Conversion1 : DataTypeConversion  SaturateOnIntegerOverflow=off  RndMeth=Floor
  First 5 Percent : simulink/Logic and Bit Operations/Compare To Constant  relop=<=  const=max(Maneuver.Trajectory.xTrajectory.Value)*0.05  OutDataTypeStr=boolean  ZeroCross=off
  Last 5 Percent : simulink/Logic and Bit Operations/Compare To Constant  relop=>=  const=max(Maneuver.Trajectory.xTrajectory.Value)*0.95  OutDataTypeStr=boolean  ZeroCross=off
  Memory : Memory  InitialCondition=false
  Memory2 : Memory  InitialCondition=false
  OR : Logic  Operator=OR  IconShape=distinctive  AllPortsSameDT=off  OutDataTypeStr=boolean
  Sum : Sum  Inputs=+-|
  Triggered Subsystem : Subsystem  TreatAsAtomicUnit=on
  Lap Count : Outport  VectorParamsAs1DForOutWhenUnconnected=off
  wires:
  Data Type Conversion1/1 -> Sum/2
  Data Type Conversion/1 -> Sum/1
  ad/1 -> First 5 Percent/1, Last 5 Percent/1
  Last 5 Percent/1 -> AND Subtract Lap/2, Memory/1  "Last 5"
  Triggered Subsystem/1(Num Laps) -> Lap Count/1
  First 5 Percent/1 -> Memory2/1, AND Add Lap/2  "First 5"
  Memory/1 -> AND Add Lap/1
  OR/1 -> Triggered Subsystem/Trigger  "Trigger"
  Memory2/1 -> AND Subtract Lap/1
  AND Add Lap/1 -> Data Type Conversion/1, OR/1  "Add Lap"
  AND Subtract Lap/1 -> OR/2, Data Type Conversion1/1  "Subtract Lap"
  Sum/1 -> Triggered Subsystem/1(Up Down)  "Counter"

== system sm_car_/Driver/Closed Loop/Maneuver/PoseTargetVisual/Pace Car ==
  Left Face : sm_lib/Body Elements/Extruded Solid  ExtrusionType=General  PolygonNumSides=3  PolygonOuterRadius=1  PolygonOuterRadiusUnits=m  ExportEntireGeometry=off  ExtrusionCrossSection=xy_data_car_side  ExtrusionCrossSectionUnits=m  ExportConvexHullGeometry=off  ExtrusionLength=thk_side  ExtrusionLengthUnits=m  InertiaType=PointMass  BasedOnType=Density  Density=1000  DensityUnits=kg/m^3  Mass=0  MassUnits=kg  CenterOfMass=[0 0 0]  CenterOfMassUnits=m  MomentsOfInertia=[1 1 1]  MomentsOfInertiaUnits=kg*m^2  ProductsOfInertia=[0 0 0]  ProductsOfInertiaUnits=kg*m^2  GraphicType=FromGeometry  MarkerShape=Sphere  MarkerSize=10  GraphicVisPropType=SimpleVisualProperties  GraphicDiffuseColor=clr_body_geo_left  GraphicOpacity=opc_body_geo_left  GraphicSpecularColor=[0.5 0.5 0.5 1.0]  GraphicAmbientColor=[0.15 0.15 0.15 1.0]  GraphicEmissiveColor=[0.0 0.0 0.0 1.0]  GraphicShininess=75  DoExposeReferenceFrame=on  SerializedFrames=<Frames/>
  Ornament Front : sm_lib/Body Elements/Extruded Solid  ExtrusionType=General  PolygonNumSides=3  PolygonOuterRadius=1  PolygonOuterRadiusUnits=m  ExportEntireGeometry=off  ExtrusionCrossSection=extr_data_emblem_f  ExtrusionCrossSectionUnits=m  ExportConvexHullGeometry=off  ExtrusionLength=0.01  ExtrusionLengthUnits=m  InertiaType=CalculateFromGeometry  BasedOnType=Density  Density=1000  DensityUnits=kg/m^3  Mass=1  MassUnits=kg  CenterOfMass=[0 0 0]  CenterOfMassUnits=m  MomentsOfInertia=[1 1 1]  MomentsOfInertiaUnits=kg*m^2  ProductsOfInertia=[0 0 0]  ProductsOfInertiaUnits=kg*m^2  GraphicType=FromGeometry  MarkerShape=Sphere  MarkerSize=10  GraphicVisPropType=SimpleVisualProperties  GraphicDiffuseColor=clr_emblem_f  GraphicOpacity=opc_emblem_f  GraphicSpecularColor=[0.5 0.5 0.5 1.0]  GraphicAmbientColor=[0.15 0.15 0.15 1.0]  GraphicEmissiveColor=[0.0 0.0 0.0 1.0]  GraphicShininess=75  DoExposeReferenceFrame=on  SerializedFrames=<Frames/>
  Ornament Rear : sm_lib/Body Elements/Extruded Solid  ExtrusionType=General  PolygonNumSides=3  PolygonOuterRadius=1  PolygonOuterRadiusUnits=m  ExportEntireGeometry=off  ExtrusionCrossSection=extr_data_emblem_r  ExtrusionCrossSectionUnits=m  ExportConvexHullGeometry=off  ExtrusionLength=0.01  ExtrusionLengthUnits=m  InertiaType=CalculateFromGeometry  BasedOnType=Density  Density=1000  DensityUnits=kg/m^3  Mass=1  MassUnits=kg  CenterOfMass=[0 0 0]  CenterOfMassUnits=m  MomentsOfInertia=[1 1 1]  MomentsOfInertiaUnits=kg*m^2  ProductsOfInertia=[0 0 0]  ProductsOfInertiaUnits=kg*m^2  GraphicType=FromGeometry  MarkerShape=Sphere  MarkerSize=10  GraphicVisPropType=SimpleVisualProperties  GraphicDiffuseColor=clr_emblem_r  GraphicOpacity=opc_emblem_r  GraphicSpecularColor=[0.5 0.5 0.5 1.0]  GraphicAmbientColor=[0.15 0.15 0.15 1.0]  GraphicEmissiveColor=[0.0 0.0 0.0 1.0]  GraphicShininess=75  DoExposeReferenceFrame=on  SerializedFrames=<Frames/>
  Rear View : sm_lib/Frames and Transforms/Reference Frame
  Right Face : sm_lib/Body Elements/Extruded Solid  ExtrusionType=General  PolygonNumSides=3  PolygonOuterRadius=1  PolygonOuterRadiusUnits=m  ExportEntireGeometry=off  ExtrusionCrossSection=xy_data_car_side  ExtrusionCrossSectionUnits=m  ExportConvexHullGeometry=off  ExtrusionLength=thk_side  ExtrusionLengthUnits=m  InertiaType=PointMass  BasedOnType=Density  Density=1000  DensityUnits=kg/m^3  Mass=0  MassUnits=kg  CenterOfMass=[0 0 0]  CenterOfMassUnits=m  MomentsOfInertia=[1 1 1]  MomentsOfInertiaUnits=kg*m^2  ProductsOfInertia=[0 0 0]  ProductsOfInertiaUnits=kg*m^2  GraphicType=FromGeometry  MarkerShape=Sphere  MarkerSize=10  GraphicVisPropType=SimpleVisualProperties  GraphicDiffuseColor=clr_body_geo_right  GraphicOpacity=opc_body_geo_right  GraphicSpecularColor=[0.5 0.5 0.5 1.0]  GraphicAmbientColor=[0.15 0.15 0.15 1.0]  GraphicEmissiveColor=[0.0 0.0 0.0 1.0]  GraphicShininess=75  DoExposeReferenceFrame=on  SerializedFrames=<Frames/>
  Top Surface : sm_lib/Body Elements/Extruded Solid  ExtrusionType=General  PolygonNumSides=3  PolygonOuterRadius=1  PolygonOuterRadiusUnits=m  ExportEntireGeometry=off  ExtrusionCrossSection=xy_data_car_top  ExtrusionCrossSectionUnits=m  ExportConvexHullGeometry=off  ExtrusionLength=car_track  ExtrusionLengthUnits=m  InertiaType=PointMass  BasedOnType=Density  Density=0  DensityUnits=kg/m^3  Mass=0  MassUnits=kg  CenterOfMass=[0 0 0]  CenterOfMassUnits=m  MomentsOfInertia=[1 1 1]  MomentsOfInertiaUnits=kg*m^2  ProductsOfInertia=[0 0 0]  ProductsOfInertiaUnits=kg*m^2  GraphicType=FromGeometry  MarkerShape=Sphere  MarkerSize=10  GraphicVisPropType=SimpleVisualProperties  GraphicDiffuseColor=clr_body_geo_top  GraphicOpacity=opc_body_geo_top  GraphicSpecularColor=[0.5 0.5 0.5 1.0]  GraphicAmbientColor=[0.15 0.15 0.15 1.0]  GraphicEmissiveColor=[0.0 0.0 0.0 1.0]  GraphicShininess=75  DoExposeReferenceFrame=on  SerializedFrames=<Frames/>
  Transform Extrusion Axes : sm_lib/Frames and Transforms/Rigid Transform  RotationMethod=StandardAxis  FollAlignAxisA=+X  BaseAlignAxisA=+Y  FollAlignAxisB=+Y  BaseAlignAxisB=+Z  RotationStandardAxis=+X  RotationAngle=90  RotationAngleUnits=deg  RotationArbitraryAxis=[0 0 1]  RotationSequenceAxes=FollowerAxes  RotationSequence=XYX  RotationSequenceAngles=[0 0 0]  RotationSequenceAnglesUnits=deg  RotationMatrix=[1 0 0; 0 1 0; 0 0 1]  Quaternion=[1 0 0 0]  TranslationMethod=None  TranslationCartesianOffset=[0 0 0]  TranslationCartesianOffsetUnits=m  TranslationStandardAxis=+Z  TranslationStandardOffset=0  TranslationStandardOffsetUnits=m  TranslationROffset=0  TranslationROffsetUnits=m  TranslationThetaOffset=0  TranslationThetaOffsetUnits=deg  TranslationZOffset=0  TranslationZOffsetUnits=m
  Transform Ornament Front : sm_lib/Frames and Transforms/Rigid Transform  RotationMethod=RotationSequence  FollAlignAxisA=+X  BaseAlignAxisA=+Y  FollAlignAxisB=+Y  BaseAlignAxisB=+Z  RotationStandardAxis=+Z  RotationAngle=90  RotationAngleUnits=deg  RotationArbitraryAxis=[0 0 1]  RotationSequenceAxes=FollowerAxes  RotationSequence=ZXY  RotationSequenceAngles=[90 90 0]  RotationSequenceAnglesUnits=deg  RotationMatrix=[1 0 0; 0 1 0; 0 0 1]  Quaternion=[1 0 0 0]  TranslationMethod=Cartesian  TranslationCartesianOffset=[max(xy_data_car_side(:,1)) 0 min(xy_data_car_side(:,2))+0.15]  TranslationCartesianOffsetUnits=m  TranslationStandardAxis=+Z  TranslationStandardOffset=1  TranslationStandardOffsetUnits=m  TranslationROffset=0  TranslationROffsetUnits=m  TranslationThetaOffset=0  TranslationThetaOffsetUnits=deg  TranslationZOffset=0  TranslationZOffsetUnits=m
  Transform Ornament Rear : sm_lib/Frames and Transforms/Rigid Transform  RotationMethod=RotationSequence  FollAlignAxisA=+X  BaseAlignAxisA=+Y  FollAlignAxisB=+Y  BaseAlignAxisB=+Z  RotationStandardAxis=+Z  RotationAngle=90  RotationAngleUnits=deg  RotationArbitraryAxis=[0 0 1]  RotationSequenceAxes=FollowerAxes  RotationSequence=ZXY  RotationSequenceAngles=[90 90 180]  RotationSequenceAnglesUnits=deg  RotationMatrix=[1 0 0; 0 1 0; 0 0 1]  Quaternion=[1 0 0 0]  TranslationMethod=Cartesian  TranslationCartesianOffset=[min(xy_data_car_side(:,1))+0.1 0 min(xy_data_car_side(:,2))+0.15]  TranslationCartesianOffsetUnits=m  TranslationStandardAxis=+Z  TranslationStandardOffset=1  TranslationStandardOffsetUnits=m  TranslationROffset=0  TranslationROffsetUnits=m  TranslationThetaOffset=0  TranslationThetaOffsetUnits=deg  TranslationZOffset=0  TranslationZOffsetUnits=m
  Transform Rear View : sm_lib/Frames and Transforms/Rigid Transform  RotationMethod=None  FollAlignAxisA=+X  BaseAlignAxisA=+Y  FollAlignAxisB=+Y  BaseAlignAxisB=+Z  RotationStandardAxis=+Z  RotationAngle=0.0  RotationAngleUnits=deg  RotationArbitraryAxis=[0 0 1]  RotationSequenceAxes=FollowerAxes  RotationSequence=XYX  RotationSequenceAngles=[0 0 0]  RotationSequenceAnglesUnits=deg  RotationMatrix=[1 0 0; 0 1 0; 0 0 1]  Quaternion=[1 0 0 0]  TranslationMethod=Cartesian  TranslationCartesianOffset=[min(xy_data_car_side(:,1))-4 0 min(xy_data_car_side(:,2))+1]  TranslationCartesianOffsetUnits=m  TranslationStandardAxis=+Z  TranslationStandardOffset=0  TranslationStandardOffsetUnits=m  TranslationROffset=0  TranslationROffsetUnits=m  TranslationThetaOffset=0  TranslationThetaOffsetUnits=deg  TranslationZOffset=0  TranslationZOffsetUnits=m
  Transform Reference : sm_lib/Frames and Transforms/Rigid Transform  RotationMethod=None  FollAlignAxisA=+X  BaseAlignAxisA=+Y  FollAlignAxisB=+Y  BaseAlignAxisB=+Z  RotationStandardAxis=+Z  RotationAngle=0.0  RotationAngleUnits=deg  RotationArbitraryAxis=[0 0 1]  RotationSequenceAxes=FollowerAxes  RotationSequence=XYX  RotationSequenceAngles=[0 0 0]  RotationSequenceAnglesUnits=deg  RotationMatrix=[1 0 0; 0 1 0; 0 0 1]  Quaternion=[1 0 0 0]  TranslationMethod=Cartesian  TranslationCartesianOffset=offset_ref  TranslationCartesianOffsetUnits=m  TranslationStandardAxis=+Z  TranslationStandardOffset=0  TranslationStandardOffsetUnits=m  TranslationROffset=0  TranslationROffsetUnits=m  TranslationThetaOffset=0  TranslationThetaOffsetUnits=deg  TranslationZOffset=0  TranslationZOffsetUnits=m
  Transform Left Face : sm_lib/Frames and Transforms/Rigid Transform  RotationMethod=None  FollAlignAxisA=+X  BaseAlignAxisA=+Y  FollAlignAxisB=+Y  BaseAlignAxisB=+Z  RotationStandardAxis=+Z  RotationAngle=0.0  RotationAngleUnits=deg  RotationArbitraryAxis=[0 0 1]  RotationSequenceAxes=FollowerAxes  RotationSequence=XYX  RotationSequenceAngles=[0 0 0]  RotationSequenceAnglesUnits=deg  RotationMatrix=[1 0 0; 0 1 0; 0 0 1]  Quaternion=[1 0 0 0]  TranslationMethod=StandardAxis  TranslationCartesianOffset=[0 0 0]  TranslationCartesianOffsetUnits=m  TranslationStandardAxis=-Z  TranslationStandardOffset=car_track/2-thk_side/2  TranslationStandardOffsetUnits=m  TranslationROffset=0  TranslationROffsetUnits=m  TranslationThetaOffset=0  TranslationThetaOffsetUnits=deg  TranslationZOffset=0  TranslationZOffsetUnits=m
  Transform Right Face : sm_lib/Frames and Transforms/Rigid Transform  RotationMethod=None  FollAlignAxisA=+X  BaseAlignAxisA=+Y  FollAlignAxisB=+Y  BaseAlignAxisB=+Z  RotationStandardAxis=+Z  RotationAngle=0.0  RotationAngleUnits=deg  RotationArbitraryAxis=[0 0 1]  RotationSequenceAxes=FollowerAxes  RotationSequence=XYX  RotationSequenceAngles=[0 0 0]  RotationSequenceAnglesUnits=deg  RotationMatrix=[1 0 0; 0 1 0; 0 0 1]  Quaternion=[1 0 0 0]  TranslationMethod=StandardAxis  TranslationCartesianOffset=[0 0 0]  TranslationCartesianOffsetUnits=m  TranslationStandardAxis=+Z  TranslationStandardOffset=car_track/2-thk_side/2  TranslationStandardOffsetUnits=m  TranslationROffset=0  TranslationROffsetUnits=m  TranslationThetaOffset=0  TranslationThetaOffsetUnits=deg  TranslationZOffset=0  TranslationZOffsetUnits=m
  FA : PMIOPort  Side=Right
  P : PMIOPort  Port=2  Side=Left
  connections:
  Transform Reference/LConn1 -- P/RConn1 -- FA/RConn1
  Transform Rear View/RConn1 -- Rear View/RConn1
  Transform Ornament Front/LConn1 -- Transform Ornament Rear/LConn1 -- Transform Rear View/LConn1 -- Transform Reference/RConn1 -- Transform Extrusion Axes/LConn1
  Left Face/RConn1 -- Transform Left Face/RConn1
  Transform Extrusion Axes/RConn1 -- Transform Right Face/LConn1 -- Top Surface/RConn1 -- Transform Left Face/LConn1
  Right Face/RConn1 -- Transform Right Face/RConn1
  Transform Ornament Front/RConn1 -- Ornament Front/RConn1
  Transform Ornament Rear/RConn1 -- Ornament Rear/RConn1

== system sm_car_/Driver/Closed Loop1/Maneuver/Count Lap/Triggered Subsystem ==
  Up Down : Inport
  Trigger : TriggerPort  VariantControl=Variant  ZeroCross=off
  Memory : Memory  InheritSampleTime=on
  Sum : Sum  Inputs=|++
  Num Laps : Outport  VectorParamsAs1DForOutWhenUnconnected=off
  wires:
  Memory/1 -> Sum/1
  Sum/1 -> Memory/1, Num Laps/1
  Up Down/1 -> Sum/2
